simulink model "CMG_Cluster"  (R2024a)
settings: Solver=FixedStepDiscrete  StartTime=0.0  StopTime=8  FixedStep=.001  RelTol=1e-3
settings Model: Creator=zz  LastModifiedBy=zz

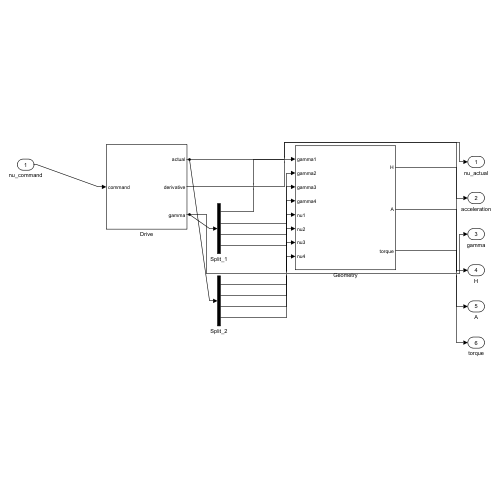
[thumbnail: Simulink's stored preview of the top-level diagram]
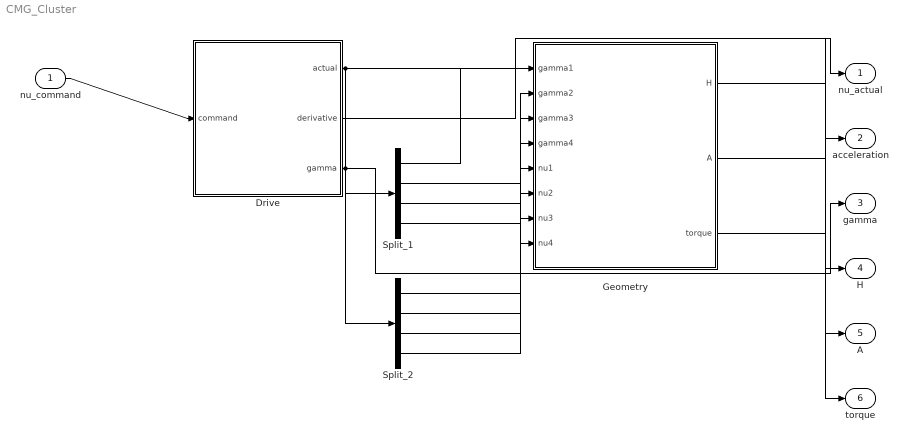
== system CMG_Cluster ==
  nu_command : Inport  PortDimensions=4
  Drive : Subsystem
  Geometry : Subsystem
  Split_1 : Demux
  Split_2 : Demux
  nu_actual : Outport
  acceleration : Outport  Port=2
  gamma : Outport  Port=3
  H : Outport  Port=4
  A : Outport  Port=5
  torque : Outport  Port=6
  wires:
  nu_command/1 -> Drive/1(command)
  Drive/3(gamma) -> Split_1/1, gamma/1
  Split_1/1 -> Geometry/1(gamma1)
  Split_1/2 -> Geometry/2(gamma2)
  Split_1/3 -> Geometry/3(gamma3)
  Split_1/4 -> Geometry/4(gamma4)
  Drive/1(actual) -> Split_2/1, nu_actual/1
  Split_2/1 -> Geometry/5(nu1)
  Split_2/2 -> Geometry/6(nu2)
  Split_2/3 -> Geometry/7(nu3)
  Split_2/4 -> Geometry/8(nu4)
  Drive/2(derivative) -> acceleration/1
  Geometry/1(H) -> H/1
  Geometry/2(A) -> A/1
  Geometry/3(torque) -> torque/1

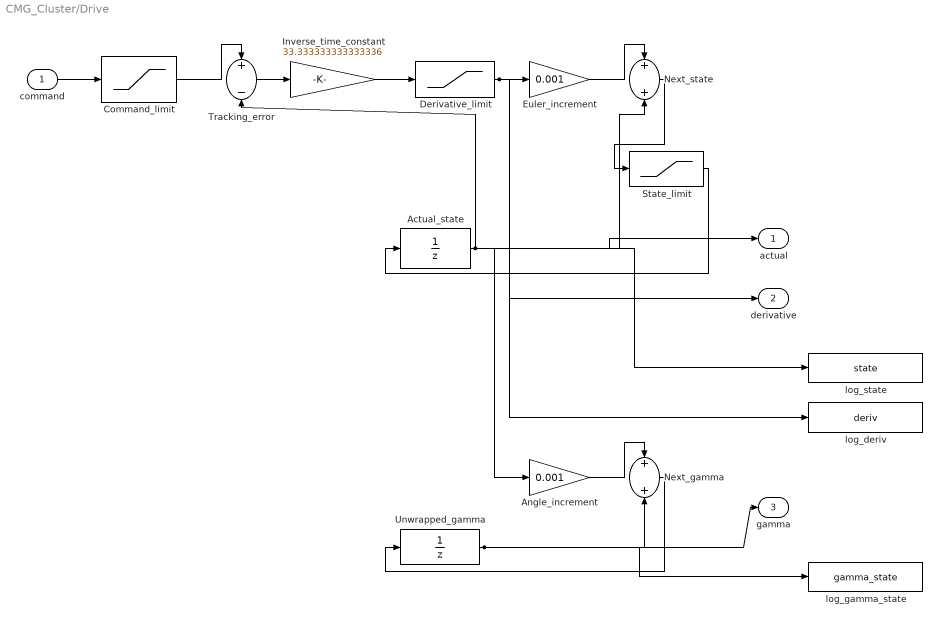
== system CMG_Cluster/Drive ==
  command : Inport  PortDimensions=4  SampleTime=0.001
  Actual_state : UnitDelay  InitialCondition=[0;0;0;0]  SampleTime=0.001
  Angle_increment : Gain  Gain=0.001
  Command_limit : Saturate  UpperLimit=[1;1;1;1]  LowerLimit=[-1;-1;-1;-1]
  Derivative_limit : Saturate  UpperLimit=[3;3;3;3]  LowerLimit=[-3;-3;-3;-3]
  Euler_increment : Gain  Gain=0.001
  Inverse_time_constant : Gain  Gain=33.333333333333336
  Next_gamma : Sum
  Next_state : Sum
  State_limit : Saturate  UpperLimit=[1;1;1;1]  LowerLimit=[-1;-1;-1;-1]
  Tracking_error : Sum  Inputs=+-
  Unwrapped_gamma : UnitDelay  InitialCondition=zeros(4,1)  SampleTime=0.001
  log_deriv : ToWorkspace  VariableName=deriv  SaveFormat=Timeseries
  log_gamma_state : ToWorkspace  VariableName=gamma_state  SaveFormat=Timeseries
  log_state : ToWorkspace  VariableName=state  SaveFormat=Timeseries
  actual : Outport
  derivative : Outport  Port=2
  gamma : Outport  Port=3
  wires:
  command/1 -> Command_limit/1
  Command_limit/1 -> Tracking_error/1
  Actual_state/1 -> Angle_increment/1, log_state/1, actual/1, Next_state/2, Tracking_error/2
  Tracking_error/1 -> Inverse_time_constant/1
  Inverse_time_constant/1 -> Derivative_limit/1
  Derivative_limit/1 -> log_deriv/1, derivative/1, Euler_increment/1
  Euler_increment/1 -> Next_state/1
  Next_state/1 -> State_limit/1
  State_limit/1 -> Actual_state/1
  Angle_increment/1 -> Next_gamma/1
  Unwrapped_gamma/1 -> log_gamma_state/1, gamma/1, Next_gamma/2
  Next_gamma/1 -> Unwrapped_gamma/1

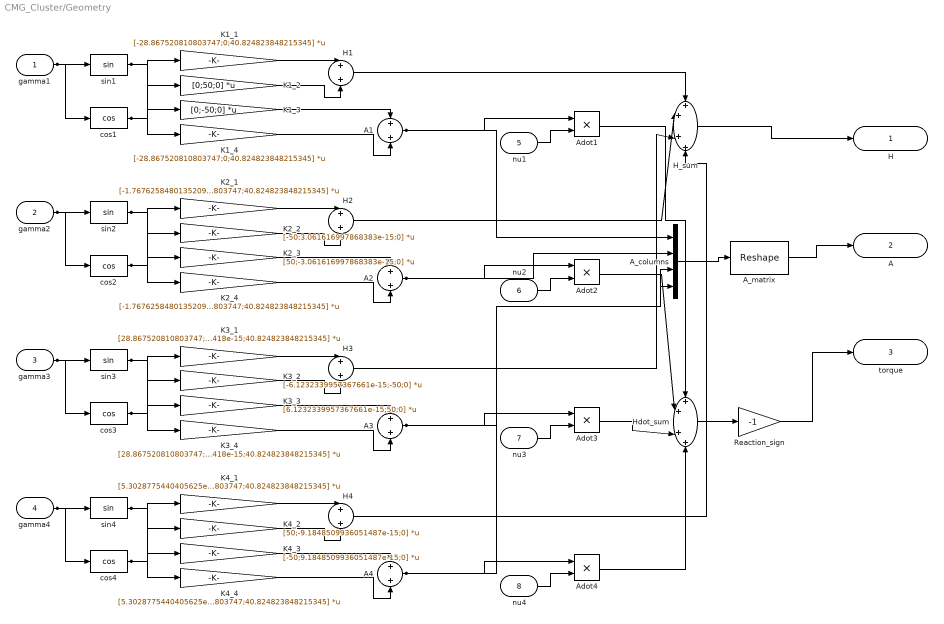
== system CMG_Cluster/Geometry ==
  gamma1 : Inport
  gamma2 : Inport  Port=2
  gamma3 : Inport  Port=3
  gamma4 : Inport  Port=4
  nu1 : Inport  Port=5
  nu2 : Inport  Port=6
  nu3 : Inport  Port=7
  nu4 : Inport  Port=8
  A{1..4} (4 alike) : Sum
  A_columns : Mux
  A_matrix : Reshape  OutputDimensionality=Customize  OutputDimensions=[3 4]
  Adot{1..4} (4 alike) : Product
  H{1..4} (4 alike) : Sum
  H_sum : Sum  Inputs=++++
  Hdot_sum : Sum  Inputs=++++
  K1_1 : Gain  Gain=[-28.867520810803747;0;40.824823848215345]  Multiplication=Matrix(K*u)
  K1_2 : Gain  Gain=[0;50;0]  Multiplication=Matrix(K*u)
  K1_3 : Gain  Gain=[0;-50;0]  Multiplication=Matrix(K*u)
  K1_4 : Gain  Gain=[-28.867520810803747;0;40.824823848215345]  Multiplication=Matrix(K*u)
  K2_1 : Gain  Gain=[-1.7676258480135209e-15;-28.867520810803747;40.824823848215345]  Multiplication=Matrix(K*u)
  K2_2 : Gain  Gain=[-50;3.061616997868383e-15;0]  Multiplication=Matrix(K*u)
  K2_3 : Gain  Gain=[50;-3.061616997868383e-15;0]  Multiplication=Matrix(K*u)
  K2_4 : Gain  Gain=[-1.7676258480135209e-15;-28.867520810803747;40.824823848215345]  Multiplication=Matrix(K*u)
  K3_1 : Gain  Gain=[28.867520810803747;-3.5352516960270418e-15;40.824823848215345]  Multiplication=Matrix(K*u)
  K3_2 : Gain  Gain=[-6.1232339957367661e-15;-50;0]  Multiplication=Matrix(K*u)
  K3_3 : Gain  Gain=[6.1232339957367661e-15;50;0]  Multiplication=Matrix(K*u)
  K3_4 : Gain  Gain=[28.867520810803747;-3.5352516960270418e-15;40.824823848215345]  Multiplication=Matrix(K*u)
  K4_1 : Gain  Gain=[5.3028775440405625e-15;28.867520810803747;40.824823848215345]  Multiplication=Matrix(K*u)
  K4_2 : Gain  Gain=[50;-9.1848509936051487e-15;0]  Multiplication=Matrix(K*u)
  K4_3 : Gain  Gain=[-50;9.1848509936051487e-15;0]  Multiplication=Matrix(K*u)
  K4_4 : Gain  Gain=[5.3028775440405625e-15;28.867520810803747;40.824823848215345]  Multiplication=Matrix(K*u)
  Reaction_sign : Gain  Gain=-1
  cos{1..4} (4 alike) : Trigonometry  Operator=cos
  sin{1..4} (4 alike) : Trigonometry
  H : Outport
  A : Outport  Port=2
  torque : Outport  Port=3
  wires:
  sin1/1 -> K1_3/1, K1_1/1
  cos1/1 -> K1_4/1, K1_2/1
  K1_1/1 -> H1/1
  K1_2/1 -> H1/2
  K1_3/1 -> A1/1
  K1_4/1 -> A1/2
  A1/1 -> A_columns/1, Adot1/1
  sin2/1 -> K2_3/1, K2_1/1
  cos2/1 -> K2_4/1, K2_2/1
  K2_1/1 -> H2/1
  K2_2/1 -> H2/2
  K2_3/1 -> A2/1
  K2_4/1 -> A2/2
  A2/1 -> A_columns/2, Adot2/1
  sin3/1 -> K3_3/1, K3_1/1
  cos3/1 -> K3_4/1, K3_2/1
  K3_1/1 -> H3/1
  K3_2/1 -> H3/2
  K3_3/1 -> A3/1
  K3_4/1 -> A3/2
  A3/1 -> A_columns/3, Adot3/1
  sin4/1 -> K4_3/1, K4_1/1
  cos4/1 -> K4_4/1, K4_2/1
  K4_1/1 -> H4/1
  K4_2/1 -> H4/2
  K4_3/1 -> A4/1
  K4_4/1 -> A4/2
  A4/1 -> A_columns/4, Adot4/1
  H1/1 -> H_sum/1
  Adot1/1 -> Hdot_sum/1
  H2/1 -> H_sum/2
  Adot2/1 -> Hdot_sum/2
  H3/1 -> H_sum/3
  Adot3/1 -> Hdot_sum/3
  H4/1 -> H_sum/4
  Adot4/1 -> Hdot_sum/4
  A_columns/1 -> A_matrix/1
  Hdot_sum/1 -> Reaction_sign/1
  gamma1/1 -> cos1/1, sin1/1
  nu1/1 -> Adot1/2
  gamma2/1 -> cos2/1, sin2/1
  nu2/1 -> Adot2/2
  gamma3/1 -> cos3/1, sin3/1
  nu3/1 -> Adot3/2
  gamma4/1 -> cos4/1, sin4/1
  nu4/1 -> Adot4/2
  H_sum/1 -> H/1
  A_matrix/1 -> A/1
  Reaction_sign/1 -> torque/1
